simulink model "sfGetStartedParallel"  (R2025b)
settings: Solver=VariableStepAuto  StartTime=0.0  StopTime=inf  RelTol=1e-3
settings Model: Creator=The MathWorks, Inc.  LastModifiedBy=The MathWorks, Inc.

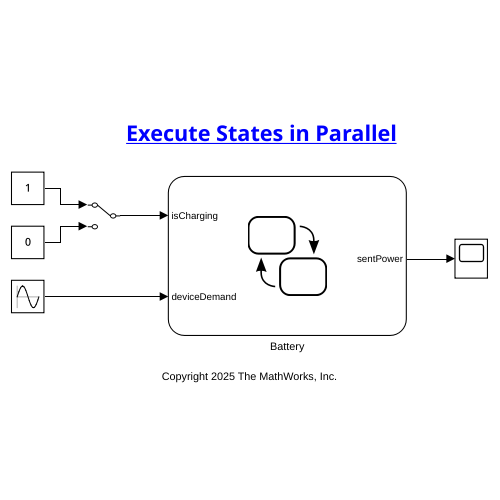
[thumbnail: Simulink's stored preview of the top-level diagram]
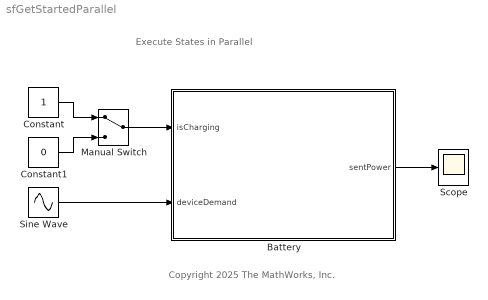
== system sfGetStartedParallel ==
  note: Copyright 2025 The MathWorks, Inc.
  note: Execute States in Parallel
  Battery : Stateflow chart  TreatAsAtomicUnit=on
  Constant : Constant
  Constant1 : Constant  Value=0
  Manual Switch : ManualSwitch
  Scope : Scope
      settings: ActiveDisplayYMinimum=-0.43749999999999989  ActiveDisplayYMaximum=3.9375
  Sine Wave : Sin  Amplitude=2.5  Bias=2.5  Phase=-pi/4  SampleTime=0
  wires:
  Manual Switch/1 -> Battery/1(isCharging)
  Constant/1 -> Manual Switch/1
  Constant1/1 -> Manual Switch/2
  Battery/1(sentPower) -> Scope/1
  Sine Wave/1 -> Battery/2(deviceDemand)

== stateflow chart sfGetStartedParallel/Battery ==
  state MainBattery
    state Charge
      entry:
      sentPower=0;
      state FastCharge
        during:
        mainCharge=mainCharge+4;
      state SlowCharge
        during:
        mainCharge=mainCharge+1;
      state Full
      (default) -> FastCharge
      FastCharge -> SlowCharge : [mainCharge>80]
      SlowCharge -> Full : [mainCharge>=100]
    state Discharge
      state Powered
        MainBattery.Discharge.Powered -> (junction 278) [order 1]
        (junction 278) -> (junction 290) [order 1] : [deviceDemand>maxPower]
        (junction 278) -> (junction 296) [order 2] : {sentPower=deviceDemand;}
        (junction 290) -> (junction 282) : {sentPower=maxPower;}
        (junction 282) -> (junction 296)
        (junction 296) -> (junction 301) : {mainCharge=mainCharge-sentPower;}
      state Empty
        entry:
        sentPower=0;
      (default) -> MainBattery.Discharge.Powered
      MainBattery.Discharge.Powered -> MainBattery.Discharge.Empty [order 1] : [mainCharge<=3]
    (default) -> Charge
    Charge -> MainBattery.Discharge : [~isCharging]
    MainBattery.Discharge -> Charge : [isCharging]
  state EmergencyBattery
    state Discharge
      state Powered
        during:
        emergencyCharge=emergencyCharge-0.01;
      state Empty
      (default) -> EmergencyBattery.Discharge.Powered
      EmergencyBattery.Discharge.Powered -> EmergencyBattery.Discharge.Empty : [emergencyCharge<=0.01]
    state Standby
    (default) -> Standby
    Standby -> EmergencyBattery.Discharge
    EmergencyBattery.Discharge -> Standby
  data: isCharging input size=1; sentPower output size=1; mainCharge local size=1 =50; deviceDemand input size=1; emergencyCharge local =100; maxPower local
